simulink model "hardwareModel_v1"  (R2025b)
settings: Solver=FixedStepAuto  StartTime=0.0  StopTime=inf  RelTol=1e-3  EnableMultiTasking=on
values from neighbouring files (symbols this model uses):
  Ts = 0.01    [modelParameters.m]
libraries: arduinomotorcarrierlib x5, arduinosensorlib x1, simulink x1, eeGeneralControl x1
settings Model: ExtModeTrigDuration=2  Creator=bkhusain  LastModifiedBy=inggi
settings SolverCC: AlgebraicLoopSolver=TrustRegion
settings OptimizationCC: EnhancedBackFolding=on  PassReuseOutputArgsThreshold=0.0  MaxStackSize=64  OptimizeBlockOrder=speed  DifferentSizesBufferReuse=on  OptimizationCustomize=off
settings DebuggingCC: ParameterTunabilityLossMsg=error  UnconnectedInputMsg=warning  UnconnectedOutputMsg=warning  UnconnectedLineMsg=warning
settings HardwareCC: ProdBitPerPointer=32.0  ProdBitPerSizeT=32.0  ProdBitPerPtrDiffT=32.0  ProdLargestAtomicInteger=Long  ProdLargestAtomicFloat=Double  ProdWordSize=32.0  ProdHWDeviceType=ARM Compatible->ARM Cortex  UseEmbeddedCoderFeatures=off  UseSimulinkCoderFeatures=off
settings ModelReferenceCC: EnableRefExpFcnMdlSchedulingChecks=on
settings SFSimCC: MATLABDynamicMemAlloc=off
settings RTWCC: SystemTargetFile=ert.tlc  HardwareBoard=Arduino Nano 33 IoT  TemplateMakefile=ert_default_tmf  Toolchain=Arduino ARM  BuildConfiguration=Faster Runs  GPUComputeCapability=3.5  Description=Embedded Coder
settings CodeAppCC: ForceParamTrailComments=on  OperatorAnnotations=on
settings ERTTargetCC: ExtModeTransport=2.0  ExtModeStaticAlloc=on  ExtModeStaticAllocSize=8192.0  ExtModeMexFile=ext_xcp  ExtModeIntrfLevel=Level2 - Open  InlinedParameterPlacement=Hierarchical  DynamicArrayContainerType=coder::array  ERTCustomFileBanners=off  SupportContinuousTime=on  SupportNonInlinedSFcns=on  RemoveResetFunc=off  SupportVariableSizeSignals=on  ModelStepFunctionPrototypeControlCompliant=off

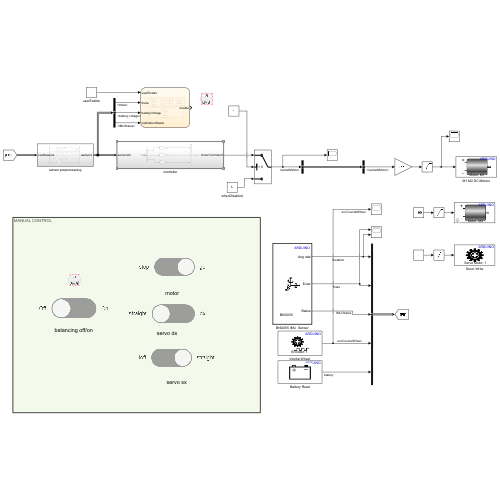
[thumbnail: Simulink's stored preview of the top-level diagram]
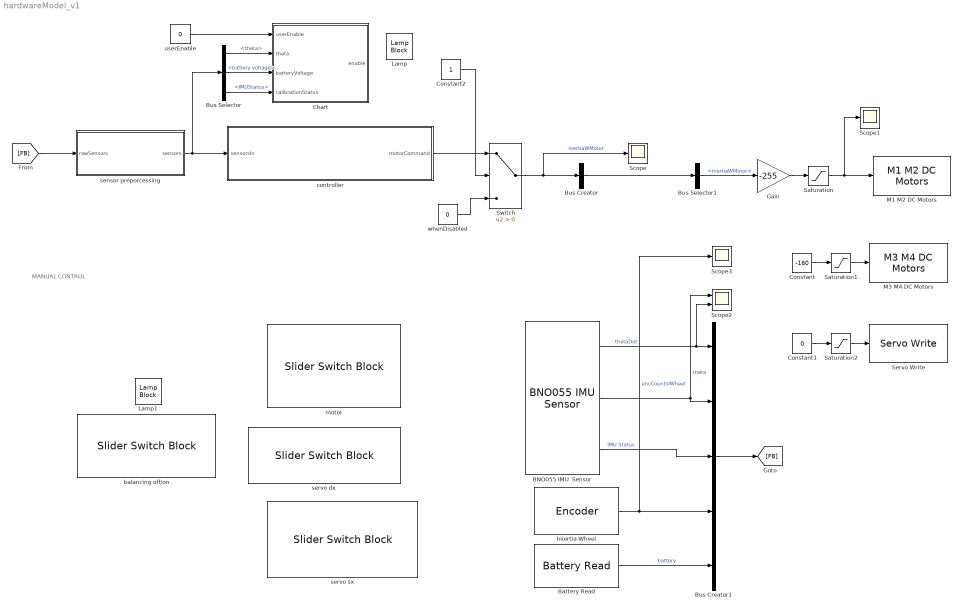
== system hardwareModel_v1 ==
  note: MANUAL CONTROL
  BNO055 IMU  Sensor : arduinosensorlib/BNO055 IMU Sensor  I2CModule=0  SlaveAddress=0x28  OperationMode=Fusion  Accel=off  AngularRate=on  MagField=off  EulerAngles=on  Quat=off  LinearAccel=off  GravityVector=off  Status=on  Timestamp=off  AccelRange=4G  AccelBW=62.5 Hz  GyroRange=2000 dps  GyroBW=32 Hz  MagODR=10 Hz  spf=1  SampleTime=Ts  blockPlatform=ARDUINO  QueueSizeFactor=1
  Battery Read : arduinomotorcarrierlib/Battery Read  SlaveAddress=uint8( hex2dec( '66' ) )  blockPlatform=ARDUINO  SampleTime=Ts
  Bus Creator : BusCreator  Inputs=1
  Bus Creator1 : BusCreator  Inputs=5
  Bus Selector : BusSelector  OutputSignals=theta,battery voltage,IMUStatus
  Bus Selector1 : BusSelector  OutputSignals=inertiaWMotor
  Chart : Stateflow chart  TreatAsAtomicUnit=on
  Constant : Constant  Value=-160
  Constant1 : Constant  Value=0
  Constant2 : Constant
  Gain : Gain  Gain=-255
  Iniertia Wheel : arduinomotorcarrierlib/Encoder  SlaveAddress=uint8( hex2dec( '66' ) )  blockPlatform=ARDUINO  Encoder=1  ShowSpeed=off  ResetOption=on  SampleTime=Ts
  Lamp : LampBlock  DefaultColor=[192.0, 192.0, 192.0]
  Lamp1 : LampBlock  DefaultColor=[192.0, 192.0, 192.0]
  M1 M2 DC Motors : arduinomotorcarrierlib/M1 M2 DC Motors  SlaveAddress=uint8( hex2dec( '66' ) )  blockPlatform=ARDUINO  MotorNumber=M1  MotorCarrierPWMFreq=100
  M3 M4 DC Motors : arduinomotorcarrierlib/M3 M4 DC Motors  MotorNumber=M4  forwardPinNumber=4  reversePinNumber=5
  Saturation : Saturate  UpperLimit=255  LowerLimit=-255
  Saturation1 : Saturate  UpperLimit=255  LowerLimit=-255
  Saturation2 : Saturate  UpperLimit=90  LowerLimit=-90
  Scope : Scope
  Scope1 : Scope
      settings: DataLoggingVariableName=ScopeData2
  Scope2 : Scope  NumInputPorts=2
      settings: DataLoggingVariableName=ScopeData3
  Scope3 : Scope
      settings: DataLoggingVariableName=ScopeData4
  Servo Write : arduinomotorcarrierlib/Servo Write  SlaveAddress=uint8( hex2dec( '66' ) )  blockPlatform=ARDUINO  MotorNumber=1  MotorCarrierPWMFreq=100
  Switch : Switch  Criteria=u2 > Threshold  SaturateOnIntegerOverflow=off  InputSameDT=off
  balancing off/on : SliderSwitchBlock  LabelPosition=Hide
  controller : Subsystem
  motor : SliderSwitchBlock  LabelPosition=Hide
  sensor preporcessing : Subsystem
  servo dx : SliderSwitchBlock  LabelPosition=Hide
  servo sx : SliderSwitchBlock  LabelPosition=Hide
  userEnable : Constant  Value=0  SampleTime=Ts
  whenDisabled : Constant  Value=0  SampleTime=Ts
  wires:
  userEnable/1 -> Chart/1(userEnable)
  [FB] -> sensor preporcessing/1(rawSensors)
  Bus Selector/1 -> Chart/2(theta)  "<theta>"
  Bus Selector/2 -> Chart/3(batteryVoltage)  "<battery voltage>"
  Switch/1 -> Scope/1, Bus Creator/1  "inertiaWMotor"
  controller/1(motorCommand) -> Switch/1
  sensor preporcessing/1(sensors) -> Bus Selector/1, controller/1(sensorsIn)
  whenDisabled/1 -> Switch/3
  Bus Selector/3 -> Chart/4(calibrationStatus)  "<IMUStatus>"
  BNO055 IMU  Sensor/3 -> Bus Creator1/3  "IMU Status"
  BNO055 IMU  Sensor/1 -> Scope2/2, Bus Creator1/1  "thetaDot"
  BNO055 IMU  Sensor/2 -> Bus Creator1/2, Scope2/1  "theta"
  Gain/1 -> Saturation/1
  Bus Creator1/1 -> [FB]
  Saturation/1 -> M1 M2 DC Motors/1, Scope1/1
  Bus Selector1/1 -> Gain/1  "<inertiaWMotor>"
  Battery Read/1 -> Bus Creator1/5  "battery"
  Bus Creator/1 -> Bus Selector1/1
  Iniertia Wheel/1 -> Scope3/1, Bus Creator1/4  "encCountsIWheel"
  Constant/1 -> Saturation1/1
  Constant1/1 -> Saturation2/1
  Saturation1/1 -> M3 M4 DC Motors/1
  Saturation2/1 -> Servo Write/1
  Constant2/1 -> Switch/2

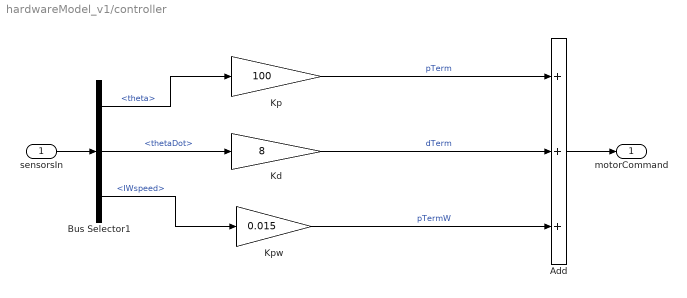
== system hardwareModel_v1/controller ==
  sensorsIn : Inport
  Add : Sum  Inputs=+++
  Bus Selector1 : BusSelector  OutputSignals=theta,thetaDot,IWspeed
  Kd : Gain  Gain=8
  Kp : Gain  Gain=100
  Kpw : Gain  Gain=0.015
  motorCommand : Outport
  wires:
  Bus Selector1/3 -> Kpw/1  "<IWspeed>"
  Kpw/1 -> Add/3  "pTermW"
  Kd/1 -> Add/2  "dTerm"
  Bus Selector1/2 -> Kd/1  "<thetaDot>"
  Bus Selector1/1 -> Kp/1  "<theta>"
  Kp/1 -> Add/1  "pTerm"
  sensorsIn/1 -> Bus Selector1/1
  Add/1 -> motorCommand/1

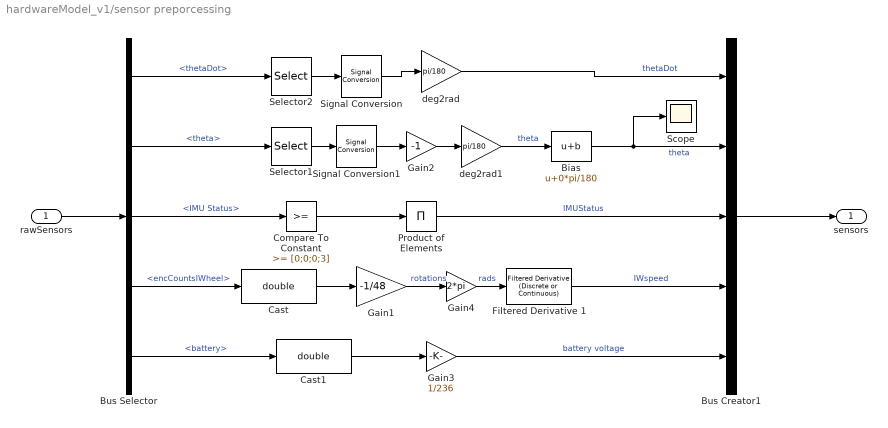
== system hardwareModel_v1/sensor preporcessing ==
  rawSensors : Inport
  Bias : Bias  Bias=0*pi/180  SaturateOnIntegerOverflow=off
  Bus Creator1 : BusCreator  Inputs=5
  Bus Selector : BusSelector  OutputSignals=thetaDot,theta,IMU Status,encCountsIWheel,battery
  Cast : DataTypeConversion  OutDataTypeStr=double  SaturateOnIntegerOverflow=off  RndMeth=Floor
  Cast1 : DataTypeConversion  OutDataTypeStr=double  SaturateOnIntegerOverflow=off  RndMeth=Floor
  Compare To Constant : simulink/Logic and Bit Operations/Compare To Constant  relop=>=  const=[0;0;0;3]  OutDataTypeStr=boolean
  Filtered Derivative 1 : eeGeneralControl/Filtered Derivative (Discrete or Continuous)  K=1  T=0.1  B=inf  A=-inf  minRatio=10  init_option=Inherited from block input  x0=0  Ts=Ts
  Gain1 : Gain  Gain=-1/48
  Gain2 : Gain  Gain=-1
  Gain3 : Gain  Gain=1/236
  Gain4 : Gain  Gain=2*pi
  Product of Elements : Product  Inputs=*
  Scope : Scope
      settings: ActiveDisplayYMinimum=-0.42289  ActiveDisplayYMaximum=-0.22289
  Selector1 : Selector  InputPortWidth=3  IndexOptions=Index vector (dialog)  Indices=[2]  OutputSizes=1
  Selector2 : Selector  InputPortWidth=3  IndexOptions=Index vector (dialog)  Indices=[2]  OutputSizes=1
  Signal Conversion : SignalConversion  OverrideOpt=off
  Signal Conversion1 : SignalConversion  OverrideOpt=off
  deg2rad : Gain  Gain=pi/180
  deg2rad1 : Gain  Gain=pi/180
  sensors : Outport
  wires:
  Bus Selector/4 -> Cast/1  "<encCountsIWheel>"
  Compare To Constant/1 -> Product of Elements/1
  Bus Selector/5 -> Cast1/1  "<battery>"
  Selector2/1 -> Signal Conversion/1
  Bus Selector/2 -> Selector1/1  "<theta>"
  Selector1/1 -> Signal Conversion1/1
  Cast1/1 -> Gain3/1
  Bus Selector/3 -> Compare To Constant/1  "<IMU Status>"
  rawSensors/1 -> Bus Selector/1
  Product of Elements/1 -> Bus Creator1/3  "IMUStatus"
  Filtered Derivative 1/1 -> Bus Creator1/4  "IWspeed"
  deg2rad1/1 -> Bias/1  "theta"
  Bus Selector/1 -> Selector2/1  "<thetaDot>"
  Gain3/1 -> Bus Creator1/5  "battery voltage"
  Bus Creator1/1 -> sensors/1
  Signal Conversion1/1 -> Gain2/1
  Gain2/1 -> deg2rad1/1
  Signal Conversion/1 -> deg2rad/1
  Cast/1 -> Gain1/1
  Gain1/1 -> Gain4/1  "rotations"
  Gain4/1 -> Filtered Derivative 1/1  "rads"
  deg2rad/1 -> Bus Creator1/1  "thetaDot"
  Bias/1 -> Scope/1, Bus Creator1/2  "theta"

== stateflow chart hardwareModel_v1/Chart ==
  state checkFallen [parallel]
    settings: executionOrder=1
    state fallen
      entry: upright = false
    state standing
      entry: upright = true
    (default) -> fallen
    fallen -> standing : [abs(theta) <pi*12/180]
    standing -> fallen : [abs(theta) > pi*12/180]
  state checkIMUCalib [parallel]
    settings: executionOrder=2
    state imuNotCalibrated
      entry:
      IMUCalibrated = false;
    state imuCalibrated
      entry:
      IMUCalibrated = true;
    (default) -> imuNotCalibrated
    imuNotCalibrated -> imuCalibrated : [calibrationStatus == true]
  state checkBattery [parallel]
    settings: executionOrder=3
    state batteryNotCharged
      entry:
      batteryOK = false;
    state batteryCharged
      entry:
      batteryOK = true;
    (default) -> batteryNotCharged
    batteryCharged -> batteryNotCharged : [batteryVoltage < 3.0]
    batteryNotCharged -> batteryCharged : [batteryVoltage >= 3.0]
  state calculateEnable [parallel]
    settings: executionOrder=4
    state disableControl
      entry: enable = false
    state enableControl
      entry: enable = true
    (default) -> disableControl
    disableControl -> enableControl : [userEnable&& batteryOK && IMUCalibrated && upright]
    enableControl -> disableControl : [not(userEnable) || not(batteryOK) || not(IMUCalibrated) || not(upright)]
  data: userEnable input; theta input; enable output; batteryVoltage input; calibrationStatus input; upright local; IMUCalibrated local; batteryOK local
